simulink model "efeitosDeAmostragem"  (R2025a)
settings: Solver=VariableStepAuto  StartTime=0.0  StopTime=inf  MaxStep=1e-5  RelTol=1e-3
libraries: dspsnks4 x1
settings Model: Creator=merisio  LastModifiedBy=merisio

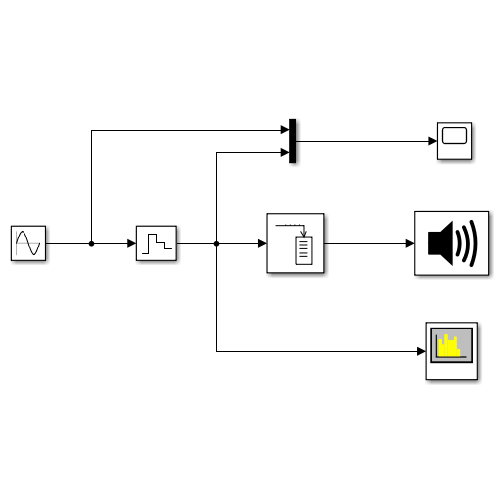
[thumbnail: Simulink's stored preview of the top-level diagram]
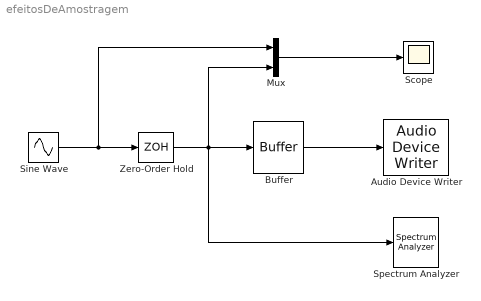
== system efeitosDeAmostragem ==
  Audio Device Writer : dspsnks4/Audio Device Writer  Driver=DirectSound  Device=Default  InheritSampleRate=on  SampleRate=44100  BitDepth=16-bit integer  BufferSize=4096  NumBuffers=10  DefaultOutputChannelMapping=on  OutputChannelMapping=1:2  OutputNumUnderrunSamples=off  DriverIdx=1  DeviceWarnFlag=''
  Buffer : Buffer  OutputFrames=off
  Mux : Mux  Inputs=2
  Scope : Scope
  Sine Wave : Sin  Frequency=2*pi*1000  Phase=pi/2  SampleTime=0
  Spectrum Analyzer : SpectrumAnalyzer  WindowPosition=[1.000000,41.000000,1366.000000,705.000000,]  ScopeFrameLocation=window  ViewType=Spectrum and spectrogram  PlotAsTwoSidedSpectrum=off  WindowInvariantSamplesPerUpdate=on  Span=750  CenterFrequency=375  StartFrequency=0  StopFrequency=750  ReferenceLoad=50  MaximizeAxes=On  YLimits=[-144.5801 26.7151]  ColorLimits=[-144.5801 26.7151]
  Zero-Order Hold : ZeroOrderHold  SampleTime=1/1500
  wires:
  Sine Wave/1 -> Mux/1, Zero-Order Hold/1
  Zero-Order Hold/1 -> Mux/2, Spectrum Analyzer/1, Buffer/1
  Buffer/1 -> Audio Device Writer/1
  Mux/1 -> Scope/1
